simulink model "hw4_2_2"  (R2025a)
settings: Solver=VariableStepAuto  StartTime=0.0  StopTime=10.0  RelTol=1e-3
settings Model: Creator=BCC  LastModifiedBy=BCC

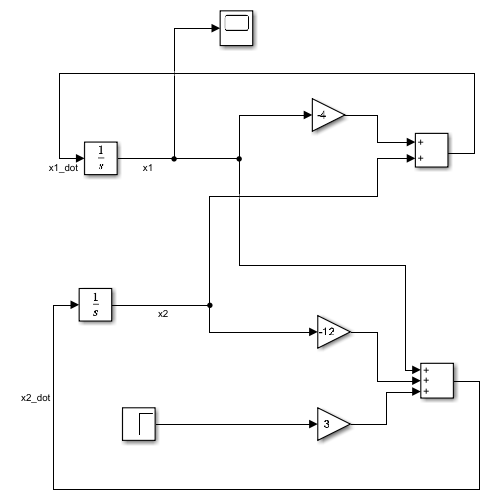
[thumbnail: Simulink's stored preview of the top-level diagram]
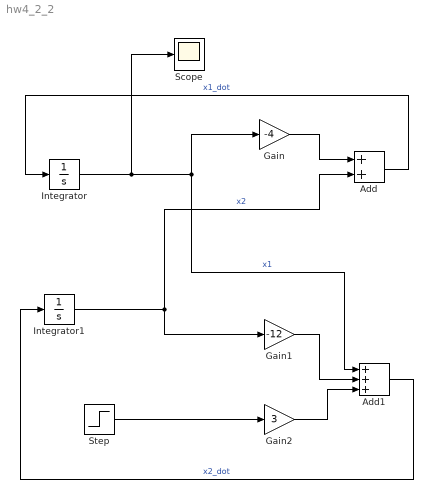
== system hw4_2_2 ==
  Add : Sum
  Add1 : Sum  Inputs=+++
  Gain : Gain  Gain=-4
  Gain1 : Gain  Gain=-12
  Gain2 : Gain  Gain=3
  Integrator : Integrator
  Integrator1 : Integrator
  Scope : Scope
      settings: ActiveDisplayYMinimum=-0.00797872340425531  ActiveDisplayYMaximum=0.071808510638297809
  Step : Step  SampleTime=0
  wires:
  Add/1 -> Integrator/1  "x1_dot"
  Integrator/1 -> Scope/1, Gain/1, Add1/1  "x1"
  Add1/1 -> Integrator1/1  "x2_dot"
  Integrator1/1 -> Add/2, Gain1/1  "x2"
  Gain/1 -> Add/1
  Step/1 -> Gain2/1
  Gain1/1 -> Add1/2
  Gain2/1 -> Add1/3
